simulink model "s4_media_distribuita"  (R2025b)
settings: Solver=ode45  StartTime=0.0  StopTime=80  FixedStep=0.002  RelTol=1e-3  EnableMultiTasking=on
settings Model: ExtModeTrigDuration=10000  Creator=sciau  LastModifiedBy=sciau
settings SolverCC: AlgebraicLoopSolver=TrustRegion  PositivePriorityOrder=on
settings DataIOCC: ReturnWorkspaceOutputs=off
settings OptimizationCC: LifeSpan=inf
settings DebuggingCC: UnconnectedInputMsg=warning  UnconnectedOutputMsg=warning  UnconnectedLineMsg=warning  ArithmeticOperatorsInVariantConditions=warning
settings ModelReferenceCC: EnableRefExpFcnMdlSchedulingChecks=on
settings SFSimCC: SimUseLocalCustomCode=off  CustomCodeUndefinedFunction=UseInterfaceOnly
settings RTWCC: SystemTargetFile=quarc_win64.tlc  TemplateMakefile=quarc_default_tmf  RTWUseLocalCustomCode=off  GPUComputeCapability=3.5  Description=QUARC Win64 Target
settings CodeAppCC: StateflowObjectComments=on
settings STFCustomTargetCC: SystemTargetFile=quarc_win64.tlc  TargetPreCompLibLocation=C:\PROGRA~3\QUARC\lib\2016a\win64\release  TargetLangStandard=C99 (ISO)  StopOnOverrun=off  Debug=off  DownloadToTarget=on
settings GRTTargetCC: ExtMode=on  ExtModeMexFile=quarc_comm  TargetPreCompLibLocation=C:\PROGRA~3\QUARC\lib\2016a\win64\release  ParMdlRefBuildCompliant=off  CompOptLevelCompliant=off  CombineOutputUpdateFcns=off  MatFileLogging=off  CPPClassGenCompliant=off  GRTInterface=on  UseToolchainInfoCompliant=off
settings ConfigComp: CovMetricSettings=dswe

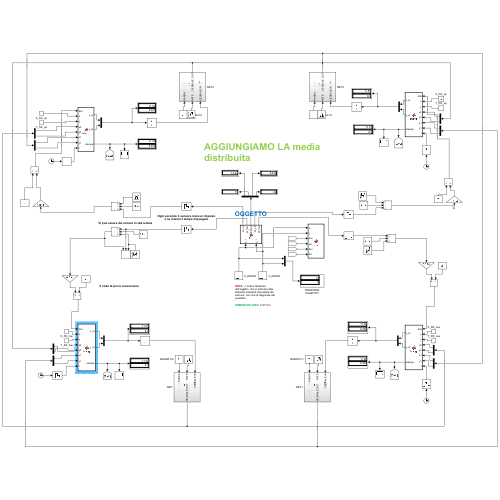
[thumbnail: Simulink's stored preview of the top-level diagram]
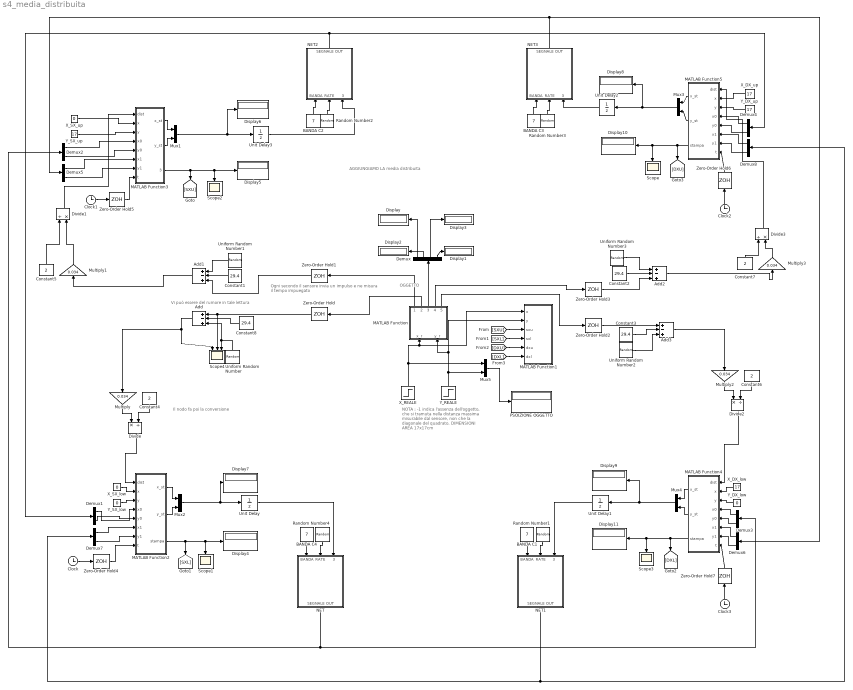
== system s4_media_distribuita ==
  note: NOTA : -1 indica l'assenza dell'oggetto, che si tramuta nella distanza massima misurabile dal sensore, non che la diagonale del quadrato.
      |
      | DIMENSIONI AREA 17x17cm
  note: OGGETTO
  note: Il nodo fa poi la conversione
  note: AGGIUNGIAMO LA media distribuita
  note: Vi può essere del rumore in tale lettura
  note: Ogni secondo il sensore invia un impulso
      | e ne misura il tempo impuegato
  Add{,1..3} (4 alike) : Sum  Inputs=+-+
  BANDA C{1..4} (4 alike) : Constant  Value=7
  Clock{,1..3} (4 alike) : Clock
  Constant{1..3,8} (4 alike) : Constant  Value=29.4
  Constant{4..7} (4 alike) : Constant  Value=2
  Demux : Demux
  Demux{1..8} (8 alike) : Demux  Outputs=2
  Display{,1..11} (12 alike) : Display
  Divide : Product  Inputs=*/
  Divide1 : Product  Inputs=/*
  Divide2 : Product  Inputs=*/
  Divide3 : Product  Inputs=/*
  MATLAB Function : MATLAB Function  TreatAsAtomicUnit=on
  MATLAB Function1 : MATLAB Function  TreatAsAtomicUnit=on
  MATLAB Function2 : MATLAB Function  TreatAsAtomicUnit=on
  MATLAB Function3 : MATLAB Function  TreatAsAtomicUnit=on
  MATLAB Function4 : MATLAB Function  TreatAsAtomicUnit=on
  MATLAB Function5 : MATLAB Function  TreatAsAtomicUnit=on
  Multiply{,1..3} (4 alike) : Gain  Gain=0.034
  Mux{1..5} (5 alike) : Mux  Inputs=2
  NET : Subsystem
  NET1 : Subsystem
  NET2 : Subsystem
  NET3 : Subsystem
  PSOIZIONE OGGETTO : Display
  Random Number1 : RandomNumber  Mean=6  Variance=6  Seed=2  SampleTime=1
  Random Number2 : RandomNumber  Mean=6  Variance=6  Seed=3  SampleTime=1
  Random Number3 : RandomNumber  Mean=6  Variance=6  Seed=4  SampleTime=1
  Random Number4 : RandomNumber  Mean=6  Variance=6  Seed=1  SampleTime=1
  Scope{,1..3} (4 alike) : Scope
      Scope settings: ActiveDisplayYMinimum=-2.3748713536925439  ActiveDisplayYMaximum=11.373842183232897
      Scope1 settings: ActiveDisplayYMinimum=-3.2499999999999996  ActiveDisplayYMaximum=19.25
      Scope2 settings: ActiveDisplayYMinimum=-1  ActiveDisplayYMaximum=1  DataLoggingVariableName=ScopeData2
      Scope3 settings: ActiveDisplayYMinimum=-2.374834675344931  ActiveDisplayYMaximum=11.37351207810438  DataLoggingVariableName=ScopeData3
  Scope4 : Scope  NumInputPorts=3
      settings: ActiveDisplayYMinimum=-77.332228841261667  ActiveDisplayYMaximum=1474.6908321791607  DataLoggingVariableName=ScopeData4
  Uniform Random Number : UniformRandomNumber  Minimum=-17.6  Maximum=17.6  SampleTime=1
  Uniform Random Number1 : UniformRandomNumber  Minimum=-0.3  Maximum=0.3  SampleTime=1
  Uniform Random Number2 : UniformRandomNumber  Minimum=-0.3  Maximum=0.3  SampleTime=1
  Uniform Random Number3 : UniformRandomNumber  Minimum=-0.3  Maximum=0.3  SampleTime=1
  Unit Delay{,1..3} (4 alike) : UnitDelay  SampleTime=-1  HasFrameUpgradeWarning=on
  X_DX_low : Constant  Value=17
  X_DX_up : Constant  Value=17
  X_REALE : Step  Before=-1  After=12  SampleTime=0
  X_SX_low : Constant  Value=0
  X_SX_up : Constant  Value=0
  Y_DX_low : Constant  Value=0
  Y_DX_up : Constant  Value=17
  Y_REALE : Step  Before=-1  After=9  SampleTime=0
  Y_SX_low : Constant  Value=0
  Y_SX_up : Constant  Value=17
  Zero-Order Hold{,1..3} (4 alike) : ZeroOrderHold
  Zero-Order Hold{4..7} (4 alike) : ZeroOrderHold  SampleTime=-1
  wires:
  MATLAB Function4/2(y_st) -> Mux4/2
  MATLAB Function2/3(stampa) -> [SXL], Scope1/1, Display4/1
  MATLAB Function5/3(stampa) -> [DXU], Scope/1, Display10/1
  Uniform Random Number3/1 -> Add2/1
  NET/1(SEGNALE OUT) -> Demux2/1, Demux3/1
  Zero-Order Hold3/1 -> Add2/3
  Constant6/1 -> Divide2/2
  Demux5/1 -> MATLAB Function3/6(x1)
  Add/1 -> Multiply/1, Scope4/1
  Mux2/1 -> Unit Delay/1, Display7/1
  Random Number3/1 -> NET3/2(RATE)
  Constant2/1 -> Add2/2
  MATLAB Function4/3(stampa) -> [DXL], Scope3/1, Display11/1
  BANDA C3/1 -> NET3/1(BANDA)
  Random Number1/1 -> NET1/2(RATE)
  MATLAB Function3/3(stampa) -> [SXU], Scope2/1, Display5/1
  Unit Delay3/1 -> NET2/3(SEGNALE IN)
  MATLAB Function/4(dx_up) -> Zero-Order Hold3/1
  NET3/1(SEGNALE OUT) -> Demux6/1, Demux5/1
  Uniform Random Number1/1 -> Add1/1
  MATLAB Function4/1(x_st) -> Mux4/1
  Unit Delay1/1 -> NET1/3(SEGNALE IN)
  Demux7/2 -> MATLAB Function2/7(y1)
  Mux1/1 -> Display6/1, Unit Delay3/1
  Constant8/1 -> Add/2
  MATLAB Function2/2(y_st) -> Mux2/2
  NET2/1(SEGNALE OUT) -> Demux4/1, Demux1/1
  Unit Delay2/1 -> NET3/3(SEGNALE IN)
  BANDA C2/1 -> NET2/1(BANDA)
  Random Number4/1 -> NET/2(RATE)
  Random Number2/1 -> NET2/2(RATE)
  NET1/1(SEGNALE OUT) -> Demux8/1, Demux7/1
  X_SX_low/1 -> MATLAB Function2/2(x)
  X_REALE/1 -> MATLAB Function/1(x_r), MATLAB Function1/1(x), Mux5/1
  Demux3/1 -> MATLAB Function4/4(x0)
  MATLAB Function5/1(x_st) -> Mux3/1
  Zero-Order Hold/1 -> Scope4/2, Add/1
  Zero-Order Hold4/1 -> MATLAB Function2/8(t)
  MATLAB Function3/1(x_st) -> Mux1/1
  Demux4/2 -> MATLAB Function5/5(y0)
  Demux8/2 -> MATLAB Function5/7(y1)
  [DXU] -> MATLAB Function1/5(dxu)
  Add2/1 -> Multiply3/1
  Demux1/2 -> MATLAB Function2/5(y0)
  Y_SX_up/1 -> MATLAB Function3/3(y)
  BANDA C1/1 -> NET1/1(BANDA)
  MATLAB Function/1(sx_up) -> Zero-Order Hold1/1
  Demux1/1 -> MATLAB Function2/4(x0)
  MATLAB Function/5(dx_low) -> Zero-Order Hold2/1
  Constant7/1 -> Divide3/1
  MATLAB Function2/1(x_st) -> Mux2/1
  Constant4/1 -> Divide/2
  Divide3/1 -> MATLAB Function5/1(dist)
  Multiply/1 -> Divide/1
  Constant5/1 -> Divide1/1
  Uniform Random Number2/1 -> Add3/3
  MATLAB Function/3(debug) -> Demux/1
  Y_DX_up/1 -> MATLAB Function5/3(y)
  MATLAB Function/2(sx_low) -> Zero-Order Hold/1
  X_DX_up/1 -> MATLAB Function5/2(x)
  Y_DX_low/1 -> MATLAB Function4/3(y)
  [SXL] -> MATLAB Function1/4(sxl)
  Demux/2 -> Display2/1
  Uniform Random Number/1 -> Add/3, Scope4/3
  Demux5/2 -> MATLAB Function3/7(y1)
  Divide/1 -> MATLAB Function2/1(dist)
  X_DX_low/1 -> MATLAB Function4/2(x)
  Multiply1/1 -> Divide1/2
  Multiply2/1 -> Divide2/1
  Mux3/1 -> Display8/1, Unit Delay2/1
  Constant3/1 -> Add3/2
  Demux6/1 -> MATLAB Function4/6(x1)
  Demux/4 -> Display1/1
  Zero-Order Hold1/1 -> Add1/3
  [SXU] -> MATLAB Function1/3(sxu)
  Demux/1 -> Display/1
  Demux/3 -> Display3/1
  Y_REALE/1 -> MATLAB Function/2(y_r), MATLAB Function1/2(y), Mux5/2
  Zero-Order Hold2/1 -> Add3/1
  Add1/1 -> Multiply1/1
  Divide2/1 -> MATLAB Function4/1(dist)
  Demux8/1 -> MATLAB Function5/6(x1)
  Demux3/2 -> MATLAB Function4/5(y0)
  Demux6/2 -> MATLAB Function4/7(y1)
  Multiply3/1 -> Divide3/2
  Demux7/1 -> MATLAB Function2/6(x1)
  MATLAB Function5/2(y_st) -> Mux3/2
  BANDA C4/1 -> NET/1(BANDA)
  Divide1/1 -> MATLAB Function3/1(dist)
  Add3/1 -> Multiply2/1
  Demux2/2 -> MATLAB Function3/5(y0)
  Mux5/1 -> PSOIZIONE OGGETTO/1
  Mux4/1 -> Unit Delay1/1, Display9/1
  MATLAB Function3/2(y_st) -> Mux1/2
  Constant1/1 -> Add1/2
  Demux2/1 -> MATLAB Function3/4(x0)
  Y_SX_low/1 -> MATLAB Function2/3(y)
  Demux4/1 -> MATLAB Function5/4(x0)
  [DXL] -> MATLAB Function1/6(dxl)
  X_SX_up/1 -> MATLAB Function3/2(x)
  Unit Delay/1 -> NET/3(SEGNALE IN)
  Clock/1 -> Zero-Order Hold4/1
  Clock1/1 -> Zero-Order Hold5/1
  Zero-Order Hold5/1 -> MATLAB Function3/8(t)
  Clock2/1 -> Zero-Order Hold6/1
  Zero-Order Hold6/1 -> MATLAB Function5/8(t)
  Clock3/1 -> Zero-Order Hold7/1
  Zero-Order Hold7/1 -> MATLAB Function4/8(t)

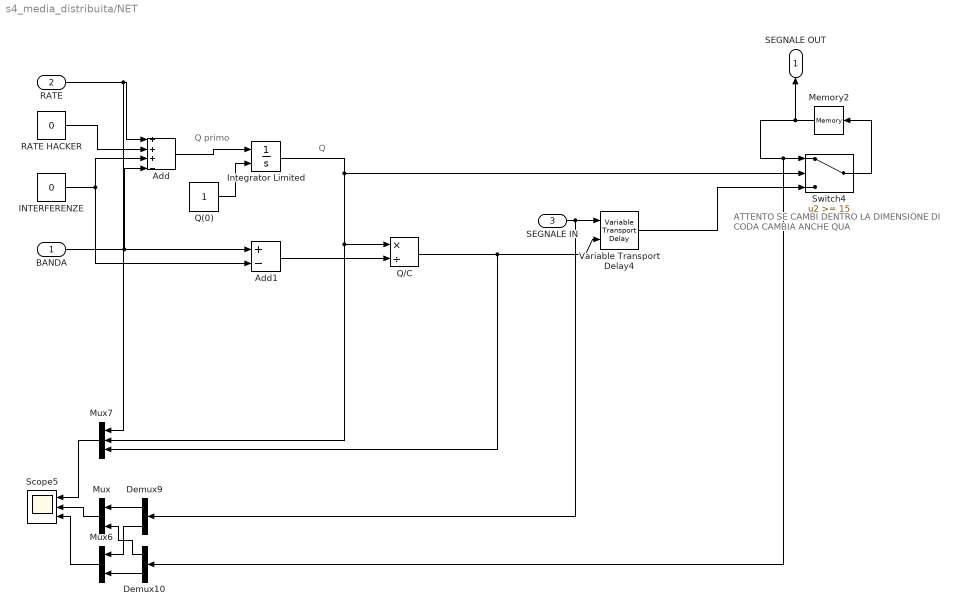
== system s4_media_distribuita/NET ==
  note: Q
  note: Q primo
  note: ATTENTO SE CAMBI
      | DENTRO LA DIMENSIONE DI CODA
      | CAMBIA ANCHE QUA
  BANDA : Inport
  RATE : Inport  Port=2
  SEGNALE IN : Inport  Port=3
  Add : Sum  Inputs=+++-
  Add1 : Sum  Inputs=+-
  Demux10 : Demux  Outputs=2
  Demux9 : Demux  Outputs=2
  INTERFERENZE : Constant  Value=0
  Integrator Limited : Integrator  InitialConditionSource=external  LimitOutput=on  UpperSaturationLimit=15  LowerSaturationLimit=0
  Memory2 : Memory
  Mux : Mux  Inputs=2
  Mux6 : Mux  Inputs=2
  Mux7 : Mux  Inputs=3
  Q(0) : Constant
  Q/C : Product  Inputs=*/
  RATE HACKER : Constant  Value=0
  Scope5 : Scope  NumInputPorts=3
      settings: ActiveDisplayYMinimum=-1  ActiveDisplayYMaximum=1  DataLoggingVariableName=ScopeData5
  Switch4 : Switch  Threshold=15  SaturateOnIntegerOverflow=off  InputSameDT=off
  Variable Transport Delay4 : VariableTransportDelay  MaximumDelay=10  ZeroDelay=on
  SEGNALE OUT : Outport
  wires:
  Add/1 -> Integrator Limited/1
  Q(0)/1 -> Integrator Limited/2
  BANDA/1 -> Add1/1, Add/4
  Add1/1 -> Q/C/2
  INTERFERENZE/1 -> Add/3, Add1/2
  RATE HACKER/1 -> Add/2
  Q/C/1 -> Mux7/3, Variable Transport Delay4/2
  Switch4/1 -> Memory2/1
  Variable Transport Delay4/1 -> Switch4/3
  Memory2/1 -> Switch4/1, Demux10/1, SEGNALE OUT/1
  Integrator Limited/1 -> Mux7/2, Q/C/1, Switch4/2
  SEGNALE IN/1 -> Variable Transport Delay4/1, Demux9/1
  RATE/1 -> Mux7/1, Add/1
  Mux/1 -> Scope5/2
  Mux7/1 -> Scope5/1
  Mux6/1 -> Scope5/3
  Demux9/2 -> Mux6/1
  Demux10/1 -> Mux/2
  Demux9/1 -> Mux/1
  Demux10/2 -> Mux6/2

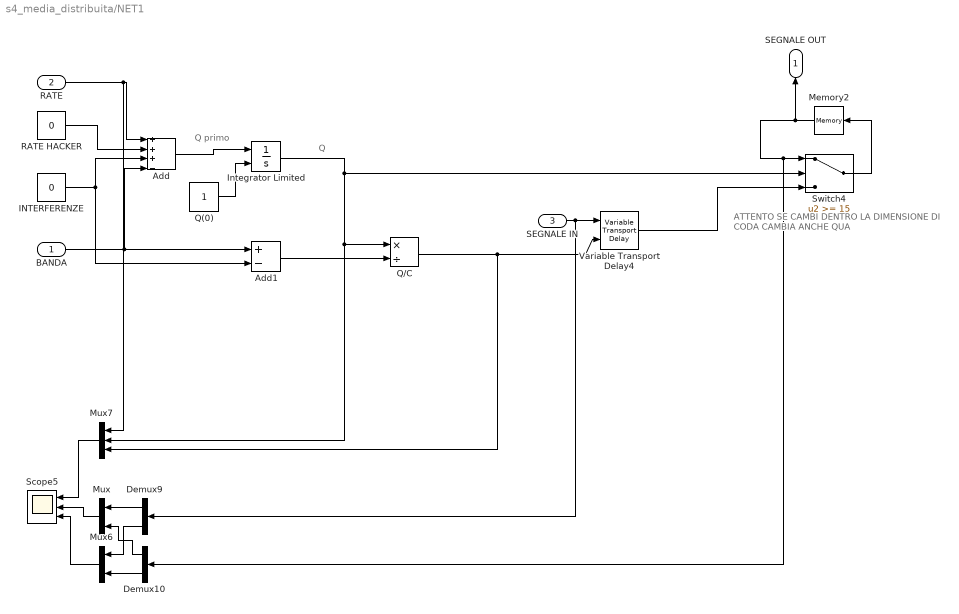
== system s4_media_distribuita/NET1 ==
  note: Q
  note: Q primo
  note: ATTENTO SE CAMBI
      | DENTRO LA DIMENSIONE DI CODA
      | CAMBIA ANCHE QUA
  BANDA : Inport
  RATE : Inport  Port=2
  SEGNALE IN : Inport  Port=3
  Add : Sum  Inputs=+++-
  Add1 : Sum  Inputs=+-
  Demux10 : Demux  Outputs=2
  Demux9 : Demux  Outputs=2
  INTERFERENZE : Constant  Value=0
  Integrator Limited : Integrator  InitialConditionSource=external  LimitOutput=on  UpperSaturationLimit=15  LowerSaturationLimit=0
  Memory2 : Memory
  Mux : Mux  Inputs=2
  Mux6 : Mux  Inputs=2
  Mux7 : Mux  Inputs=3
  Q(0) : Constant
  Q/C : Product  Inputs=*/
  RATE HACKER : Constant  Value=0
  Scope5 : Scope  NumInputPorts=3
      settings: ActiveDisplayYMinimum=-1  ActiveDisplayYMaximum=1  DataLoggingVariableName=ScopeData5
  Switch4 : Switch  Threshold=15  SaturateOnIntegerOverflow=off  InputSameDT=off
  Variable Transport Delay4 : VariableTransportDelay  MaximumDelay=10  ZeroDelay=on
  SEGNALE OUT : Outport
  wires:
  Add/1 -> Integrator Limited/1
  Q(0)/1 -> Integrator Limited/2
  BANDA/1 -> Add1/1, Add/4
  Add1/1 -> Q/C/2
  INTERFERENZE/1 -> Add/3, Add1/2
  RATE HACKER/1 -> Add/2
  Q/C/1 -> Mux7/3, Variable Transport Delay4/2
  Switch4/1 -> Memory2/1
  Variable Transport Delay4/1 -> Switch4/3
  Memory2/1 -> Switch4/1, Demux10/1, SEGNALE OUT/1
  Integrator Limited/1 -> Mux7/2, Q/C/1, Switch4/2
  SEGNALE IN/1 -> Variable Transport Delay4/1, Demux9/1
  RATE/1 -> Mux7/1, Add/1
  Mux/1 -> Scope5/2
  Mux7/1 -> Scope5/1
  Mux6/1 -> Scope5/3
  Demux9/2 -> Mux6/1
  Demux10/1 -> Mux/2
  Demux9/1 -> Mux/1
  Demux10/2 -> Mux6/2

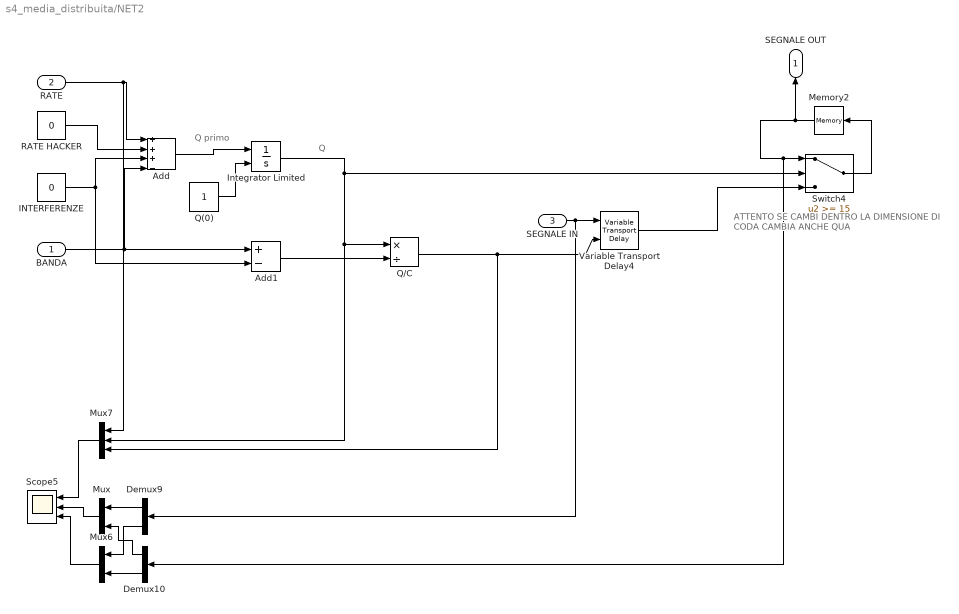
== system s4_media_distribuita/NET2 ==
  note: Q
  note: Q primo
  note: ATTENTO SE CAMBI
      | DENTRO LA DIMENSIONE DI CODA
      | CAMBIA ANCHE QUA
  BANDA : Inport
  RATE : Inport  Port=2
  SEGNALE IN : Inport  Port=3
  Add : Sum  Inputs=+++-
  Add1 : Sum  Inputs=+-
  Demux10 : Demux  Outputs=2
  Demux9 : Demux  Outputs=2
  INTERFERENZE : Constant  Value=0
  Integrator Limited : Integrator  InitialConditionSource=external  LimitOutput=on  UpperSaturationLimit=15  LowerSaturationLimit=0
  Memory2 : Memory
  Mux : Mux  Inputs=2
  Mux6 : Mux  Inputs=2
  Mux7 : Mux  Inputs=3
  Q(0) : Constant
  Q/C : Product  Inputs=*/
  RATE HACKER : Constant  Value=0
  Scope5 : Scope  NumInputPorts=3
      settings: ActiveDisplayYMinimum=-1.8749999999999996  ActiveDisplayYMaximum=16.875  DataLoggingVariableName=ScopeData5
  Switch4 : Switch  Threshold=15  SaturateOnIntegerOverflow=off  InputSameDT=off
  Variable Transport Delay4 : VariableTransportDelay  MaximumDelay=10  ZeroDelay=on
  SEGNALE OUT : Outport
  wires:
  Add/1 -> Integrator Limited/1
  Q(0)/1 -> Integrator Limited/2
  BANDA/1 -> Add1/1, Add/4
  Add1/1 -> Q/C/2
  INTERFERENZE/1 -> Add/3, Add1/2
  RATE HACKER/1 -> Add/2
  Q/C/1 -> Mux7/3, Variable Transport Delay4/2
  Switch4/1 -> Memory2/1
  Variable Transport Delay4/1 -> Switch4/3
  Memory2/1 -> Switch4/1, Demux10/1, SEGNALE OUT/1
  Integrator Limited/1 -> Mux7/2, Q/C/1, Switch4/2
  SEGNALE IN/1 -> Variable Transport Delay4/1, Demux9/1
  RATE/1 -> Mux7/1, Add/1
  Mux/1 -> Scope5/2
  Mux7/1 -> Scope5/1
  Mux6/1 -> Scope5/3
  Demux9/2 -> Mux6/1
  Demux10/1 -> Mux/2
  Demux9/1 -> Mux/1
  Demux10/2 -> Mux6/2

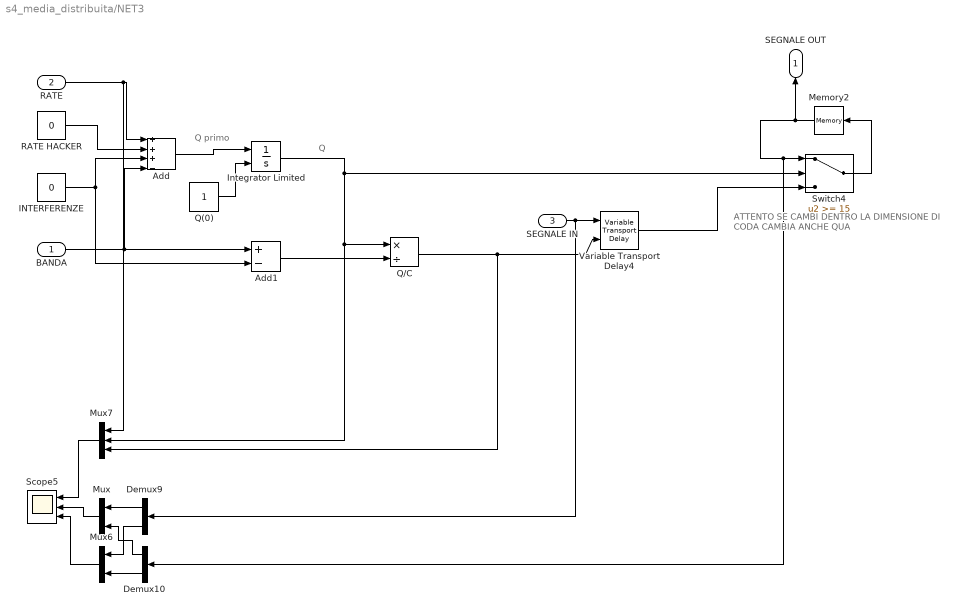
== system s4_media_distribuita/NET3 ==
  note: Q
  note: Q primo
  note: ATTENTO SE CAMBI
      | DENTRO LA DIMENSIONE DI CODA
      | CAMBIA ANCHE QUA
  BANDA : Inport
  RATE : Inport  Port=2
  SEGNALE IN : Inport  Port=3
  Add : Sum  Inputs=+++-
  Add1 : Sum  Inputs=+-
  Demux10 : Demux  Outputs=2
  Demux9 : Demux  Outputs=2
  INTERFERENZE : Constant  Value=0
  Integrator Limited : Integrator  InitialConditionSource=external  LimitOutput=on  UpperSaturationLimit=15  LowerSaturationLimit=0
  Memory2 : Memory
  Mux : Mux  Inputs=2
  Mux6 : Mux  Inputs=2
  Mux7 : Mux  Inputs=3
  Q(0) : Constant
  Q/C : Product  Inputs=*/
  RATE HACKER : Constant  Value=0
  Scope5 : Scope  NumInputPorts=3
      settings: ActiveDisplayYMinimum=-1.8749999999999996  ActiveDisplayYMaximum=16.875  DataLoggingVariableName=ScopeData5
  Switch4 : Switch  Threshold=15  SaturateOnIntegerOverflow=off  InputSameDT=off
  Variable Transport Delay4 : VariableTransportDelay  MaximumDelay=10  ZeroDelay=on
  SEGNALE OUT : Outport
  wires:
  Add/1 -> Integrator Limited/1
  Q(0)/1 -> Integrator Limited/2
  BANDA/1 -> Add1/1, Add/4
  Add1/1 -> Q/C/2
  INTERFERENZE/1 -> Add/3, Add1/2
  RATE HACKER/1 -> Add/2
  Q/C/1 -> Mux7/3, Variable Transport Delay4/2
  Switch4/1 -> Memory2/1
  Variable Transport Delay4/1 -> Switch4/3
  Memory2/1 -> Switch4/1, Demux10/1, SEGNALE OUT/1
  Integrator Limited/1 -> Mux7/2, Q/C/1, Switch4/2
  SEGNALE IN/1 -> Variable Transport Delay4/1, Demux9/1
  RATE/1 -> Mux7/1, Add/1
  Mux/1 -> Scope5/2
  Mux7/1 -> Scope5/1
  Mux6/1 -> Scope5/3
  Demux9/2 -> Mux6/1
  Demux10/1 -> Mux/2
  Demux9/1 -> Mux/1
  Demux10/2 -> Mux6/2

== matlab function s4_media_distribuita/MATLAB Function1 ==
  data: x input; y input; sxu input; sxl input; dxu input; dxl input
function dis(x,y,sxu,sxl,dxu,dxl)

    % Mantieni il grafico attivo tra le chiamate
    persistent firstRun
    if isempty(firstRun)
        firstRun = true;
    end

    % --- Disegno iniziale del quadrato (solo la prima volta) ---
    if firstRun
        clf;
        axis equal;
        grid on;
        hold on;

        % Centro del quadrato
        cx = 8.5;
        cy = 8.5;
        L = 17;

        % Vertici del quadrato
        X = [cx-L/2, cx+L/2, cx+L/2, cx-L/2, cx-L/2];
        Y = [cy-L/2, cy-L/2, cy+L/2, cy+L/2, cy-L/2];

        plot(X, Y, 'b-', 'LineWidth', 2);
        firstRun = false;
    end

    % --- Disegno dei punti SOLO quando cambiano valore ---
    if x > -1 && y > -1
        plot(x, y, 'ro', 'MarkerSize', 10, 'LineWidth', 2);
        plot(sxu(1), sxu(2), 'go', 'MarkerSize', 3, 'LineWidth', 2);
        plot(sxl(1), sxl(2), 'mo', 'MarkerSize', 6, 'LineWidth', 2);
        plot(dxu(1), dxu(2), 'co', 'MarkerSize', 9, 'LineWidth', 2);
        plot(dxl(1), dxl(2), 'yo', 'MarkerSize', 12, 'LineWidth', 2);
    end


end

== matlab function s4_media_distribuita/MATLAB Function ==
  data: x_r input; sx_up output; y_r input; sx_low output; debug output; dx_up output; dx_low output
function [sx_up, sx_low, debug, dx_up, dx_low]= fcn(x_r, y_r)

idle_dist=22;
idle_time=(idle_dist*2)/0.034;

if x_r==-1 && y_r==-1
        sx_up=idle_time;
        sx_low=idle_time;
        dx_low=idle_time;
        dx_up=idle_time;

        debug=[idle_dist,idle_dist,idle_dist,idle_dist];
else
    
    debug=[-1,-1,-1,-1];

    %sensore in (0,0)
    %0=a*0+q->q=0
    %y_r=a*x_r+0
    
    a=y_r/x_r;
    %vedo se è nel range di coefficienti angolari per cui il punto è nel
    %cono di visione

    if a>tand(30) && a<tand(60)
        cm=sqrt((0-x_r)^2+(0-y_r)^2);
        sx_low=(cm*2)/0.034;
        debug(2)=cm;
    else
        sx_low=idle_time;
        debug(2)=idle_dist;
    end
    
    

    %sensore in (17,17)
    %17=a*17+q->q=17-a*17
    %y_r=a*x_r+q=a*x_r+17-a*17
    
    a=(y_r-17)/(x_r-17);
    %vedo se è nel range di coefficienti angolari per cui il punto è nel
    %cono di visione

    if a>tand(30) && a<tand(60)
        cm=sqrt((17-x_r)^2+(17-y_r)^2);
        dx_up=(cm*2)/0.034;
        debug(3)=cm;
    else
        dx_up=idle_time;
        debug(3)=idle_dist;
    end

    

    %sensore in (0,17)
    %17=a*0+q->q=17
    %y_r=a*x_r+q=a*x_r+17
    
    a=(y_r-17)/(x_r);
    %vedo se è nel range di coefficienti angolari per cui il punto è nel
    %cono di visione

    if a>tand(120) && a<tand(150)
        cm=sqrt((0-x_r)^2+(17-y_r)^2);
        sx_up=(cm*2)/0.034;
        debug(1)=cm;
    else
        sx_up=idle_time;
        debug(1)=idle_dist;
    end

    

    %sensore in (17,0)
    %0=a*17+q->q=-a17
    %y_r=a*x_r+q=a*x_r-a17
    
    a=(y_r)/(x_r-17);
    %vedo se è nel range di coefficienti angolari per cui il punto è nel
    %cono di visione

    if a>tand(120) && a<tand(150)
        cm=sqrt((17-x_r)^2+(0-y_r)^2);
        dx_low=(cm*2)/0.034;
        debug(4)=cm;
    else
        dx_low=idle_time;
        debug(4)=idle_dist;
    end

    

end

end

== matlab function s4_media_distribuita/MATLAB Function2 ==
  data: dist input; x input; y input; x_st output; y_st output; x0 input; y0 input; x1 input; y1 input; stampa output; t input
function [x_st, y_st,stampa] = triang(dist,x,y, x0, y0,x1,y1,t)

    
    
    % persistent firstMedia
    % if isempty(firstMedia)
    %     firstMedia = true;
    % end

    persistent xst
    persistent yst;

    if isempty(xst) && isempty(yst)
        % xst=8.5;
        % yst=8.5;
        xst=0.1;
        yst=0.1;
    end

    % persistent xi
    % persistent yi;
    % 
    % if isempty(xi) && isempty(yi)
    %     % xst=8.5;
    %     % yst=8.5;
    %     xi=-1;
    %     yi=-1;
    % end
   
    if t<=40
        if dist<=20  
            x_st=xst;
            y_st=yst;
            lo_vedo=1;
        else
            x_st=-1;
            y_st=-1;
            lo_vedo=0;
        end
    
        x_medio=xst;
        y_medio=yst;
        n=1;
    
        if x0~=-1
            x_medio=x_medio+x0;
            y_medio=y_medio+y0;
            n=n+1;
        end
        if x1~=-1
            x_medio=x_medio+x1;
            y_medio=y_medio+y1;
            n=n+1;
        end
    
        x_medio=x_medio/n;
        y_medio=y_medio/n;
    
        if lo_vedo==1
            rx = x_medio-x;
            ry = y_medio-y;
            r=sqrt(rx*rx+ry*ry);
            error=r-dist;
        
            ux=rx/r;
            uy=ry/r;
        
            xst = x_medio - 0.5 * error * ux;
            yst = y_medio - 0.5 * error * uy;
        else
            xst = x_medio;
            yst = y_medio;
        end
    
        stampa=[xst,yst];
    else
        
        if x0~=-1
            xst=xst-0.5*1*(xst-x0);
            yst=yst-0.5*1*(yst-y0);
        end
        if x1~=-1
            xst=xst-0.5*1*(xst-x1);     
            yst=yst-0.5*1*(yst-y1);
        end

        x_st=xst;
        y_st=yst;

        stampa=[xst,yst];
    end


end

== matlab function s4_media_distribuita/MATLAB Function3 ==
  data: dist input; x input; y input; x_st output; y_st output; x0 input; y0 input; x1 input; y1 input; stampa output; t input
function [x_st, y_st,stampa] = triang(dist,x,y, x0, y0,x1,y1,t)

    
    
    % persistent firstMedia
    % if isempty(firstMedia)
    %     firstMedia = true;
    % end

    persistent xst
    persistent yst;

    if isempty(xst) && isempty(yst)
        % xst=8.5;
        % yst=8.5;
        xst=0.1;
        yst=0.1;
    end

    % persistent xi
    % persistent yi;
    % 
    % if isempty(xi) && isempty(yi)
    %     % xst=8.5;
    %     % yst=8.5;
    %     xi=-1;
    %     yi=-1;
    % end
   
    if t<=40
        if dist<=20  
            x_st=xst;
            y_st=yst;
            lo_vedo=1;
        else
            x_st=-1;
            y_st=-1;
            lo_vedo=0;
        end
    
        x_medio=xst;
        y_medio=yst;
        n=1;
    
        if x0~=-1
            x_medio=x_medio+x0;
            y_medio=y_medio+y0;
            n=n+1;
        end
        if x1~=-1
            x_medio=x_medio+x1;
            y_medio=y_medio+y1;
            n=n+1;
        end
    
        x_medio=x_medio/n;
        y_medio=y_medio/n;
    
        if lo_vedo==1
            rx = x_medio-x;
            ry = y_medio-y;
            r=sqrt(rx*rx+ry*ry);
            error=r-dist;
        
            ux=rx/r;
            uy=ry/r;
        
            xst = x_medio - 0.5 * error * ux;
            yst = y_medio - 0.5 * error * uy;
        else
            xst = x_medio;
            yst = y_medio;
        end
    
        stampa=[xst,yst];
    else
        
        if x0~=-1
            xst=xst-0.5*1*(xst-x0);
            yst=yst-0.5*1*(yst-y0);
        end
        if x1~=-1
            xst=xst-0.5*1*(xst-x1);     
            yst=yst-0.5*1*(yst-y1);
        end

        x_st=xst;
        y_st=yst;

        stampa=[xst,yst];
    end


end

== matlab function s4_media_distribuita/MATLAB Function4 ==
  data: dist input; x input; y input; x_st output; y_st output; x0 input; y0 input; x1 input; y1 input; stampa output; t input
function [x_st, y_st,stampa] = triang(dist,x,y, x0, y0,x1,y1,t)

    
    
    % persistent firstMedia
    % if isempty(firstMedia)
    %     firstMedia = true;
    % end

    persistent xst
    persistent yst;

    if isempty(xst) && isempty(yst)
        % xst=8.5;
        % yst=8.5;
        xst=0.1;
        yst=0.1;
    end

    % persistent xi
    % persistent yi;
    % 
    % if isempty(xi) && isempty(yi)
    %     % xst=8.5;
    %     % yst=8.5;
    %     xi=-1;
    %     yi=-1;
    % end
   
    if t<=40
        if dist<=20  
            x_st=xst;
            y_st=yst;
            lo_vedo=1;
        else
            x_st=-1;
            y_st=-1;
            lo_vedo=0;
        end
    
        x_medio=xst;
        y_medio=yst;
        n=1;
    
        if x0~=-1
            x_medio=x_medio+x0;
            y_medio=y_medio+y0;
            n=n+1;
        end
        if x1~=-1
            x_medio=x_medio+x1;
            y_medio=y_medio+y1;
            n=n+1;
        end
    
        x_medio=x_medio/n;
        y_medio=y_medio/n;
    
        if lo_vedo==1
            rx = x_medio-x;
            ry = y_medio-y;
            r=sqrt(rx*rx+ry*ry);
            error=r-dist;
        
            ux=rx/r;
            uy=ry/r;
        
            xst = x_medio - 0.5 * error * ux;
            yst = y_medio - 0.5 * error * uy;
        else
            xst = x_medio;
            yst = y_medio;
        end
    
        stampa=[xst,yst];
    else
        
        if x0~=-1
            xst=xst-0.5*1*(xst-x0);
            yst=yst-0.5*1*(yst-y0);
        end
        if x1~=-1
            xst=xst-0.5*1*(xst-x1);     
            yst=yst-0.5*1*(yst-y1);
        end

        x_st=xst;
        y_st=yst;

        stampa=[xst,yst];
    end


end

== matlab function s4_media_distribuita/MATLAB Function5 ==
  data: dist input; x input; y input; x_st output; y_st output; x0 input; y0 input; x1 input; y1 input; stampa output; t input
function [x_st, y_st,stampa] = triang(dist,x,y, x0, y0,x1,y1,t)

    
    
    % persistent firstMedia
    % if isempty(firstMedia)
    %     firstMedia = true;
    % end

    persistent xst
    persistent yst;

    if isempty(xst) && isempty(yst)
        % xst=8.5;
        % yst=8.5;
        xst=0.1;
        yst=0.1;
    end

    % persistent xi
    % persistent yi;
    % 
    % if isempty(xi) && isempty(yi)
    %     % xst=8.5;
    %     % yst=8.5;
    %     xi=-1;
    %     yi=-1;
    % end
   
    if t<=40
        if dist<=20  
            x_st=xst;
            y_st=yst;
            lo_vedo=1;
        else
            x_st=-1;
            y_st=-1;
            lo_vedo=0;
        end
    
        x_medio=xst;
        y_medio=yst;
        n=1;
    
        if x0~=-1
            x_medio=x_medio+x0;
            y_medio=y_medio+y0;
            n=n+1;
        end
        if x1~=-1
            x_medio=x_medio+x1;
            y_medio=y_medio+y1;
            n=n+1;
        end
    
        x_medio=x_medio/n;
        y_medio=y_medio/n;
    
        if lo_vedo==1
            rx = x_medio-x;
            ry = y_medio-y;
            r=sqrt(rx*rx+ry*ry);
            error=r-dist;
        
            ux=rx/r;
            uy=ry/r;
        
            xst = x_medio - 0.5 * error * ux;
            yst = y_medio - 0.5 * error * uy;
        else
            xst = x_medio;
            yst = y_medio;
        end
    
        stampa=[xst,yst];
    else
        
        if x0~=-1
            xst=xst-0.5*1*(xst-x0);
            yst=yst-0.5*1*(yst-y0);
        end
        if x1~=-1
            xst=xst-0.5*1*(xst-x1);     
            yst=yst-0.5*1*(yst-y1);
        end

        x_st=xst;
        y_st=yst;

        stampa=[xst,yst];
    end


end
